simulink model "sweep_freq"  (R2024a)
settings: Solver=FixedStepAuto  StartTime=0.0  StopTime=100  FixedStep=0.001  RelTol=1e-3
settings Model: Creator=sia429  LastModifiedBy=admin

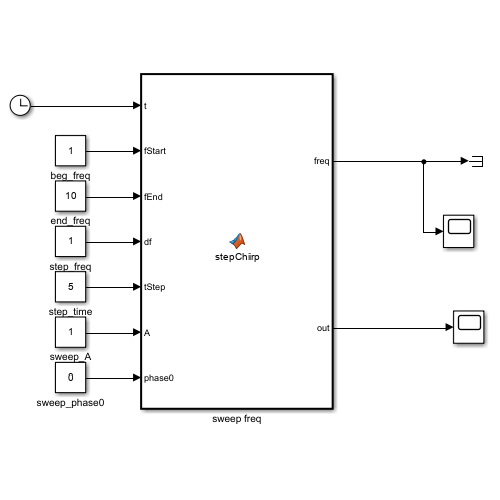
[thumbnail: Simulink's stored preview of the top-level diagram]
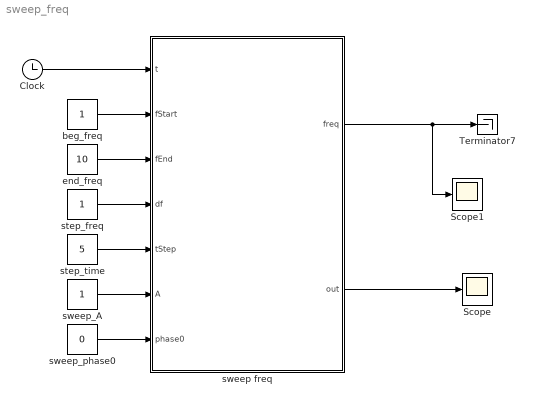
== system sweep_freq ==
  Clock : Clock
  Scope : Scope
  Scope1 : Scope
  Terminator7 : Terminator
  beg_freq : Constant  SampleTime=-1
  end_freq : Constant  Value=10  SampleTime=-1
  step_freq : Constant  SampleTime=-1
  step_time : Constant  Value=5  SampleTime=-1
  sweep freq : MATLAB Function  TreatAsAtomicUnit=on
  sweep_A : Constant  SampleTime=-1
  sweep_phase0 : Constant  Value=0  SampleTime=-1
  wires:
  step_freq/1 -> sweep freq/4(df)
  sweep_phase0/1 -> sweep freq/7(phase0)
  sweep freq/2(out) -> Scope/1
  beg_freq/1 -> sweep freq/2(fStart)
  sweep freq/1(freq) -> Scope1/1, Terminator7/1
  step_time/1 -> sweep freq/5(tStep)
  end_freq/1 -> sweep freq/3(fEnd)
  Clock/1 -> sweep freq/1(t)
  sweep_A/1 -> sweep freq/6(A)

== matlab function sweep_freq/sweep freq ==
  data: t input; fStart input; freq output; fEnd input; df input; tStep input; A input; out output; phase0 input
function [freq, out] = stepChirp(t, fStart, fEnd, df, tStep, A, phase0)

    nSeg = floor(abs(fEnd - fStart) / abs(df) + 1e-9) + 1;
    totalSweepTime = nSeg * tStep;
    
   
    if t >= totalSweepTime
        freq = 0;
        out = 0;
    else
        segIdx = floor(t / tStep);
        if segIdx >= nSeg
            segIdx = nSeg - 1;
            tInSeg = t - segIdx * tStep; 
        else
            tInSeg = t - segIdx * tStep;
        end

        freq = fStart + segIdx * df;

        phasePrev = 2*pi * ( segIdx*fStart + df*segIdx*(segIdx-1)/2 ) * tStep;
        phaseCur  = 2*pi * freq * tInSeg;
        phase = mod(phase0 + phasePrev + phaseCur, 2*pi);

        out = A * cos(phase);
    end
    



end
